simulink model "svm_dtc_winder_clean"  (R2026a)
settings: Solver=VariableStepAuto  StopTime=Tsim  MaxStep=1e-6
undefined symbols (not defined in the file): B, C_web, draw_max, draw_takeup, F0, F_ref, F_slack, ff_full, ff_on, filt_on, Fmax, h, H0, Jc, Jm, K_web, Ki_F, Ki_speed, Kp_F, Kp_speed, lambda_ref, p, r0, rc, rho, rmax, Rs, Rs_factor, T_ramp, t_rev, tau_F, Tmax, Ts_dtc, Ts_pwm, v_line_set, Vdc, w, w_max, w_min, w_ref, web_w, winder_mode_set
libraries: nesl_utility x13, fl_lib x10, ee_lib x5, slpidlib x2, eePwmGeneratorTwoLevel x1
settings Model: Creator=kunal  LastModifiedBy=kunal
settings SimscapeCC: SimscapeLogType=none

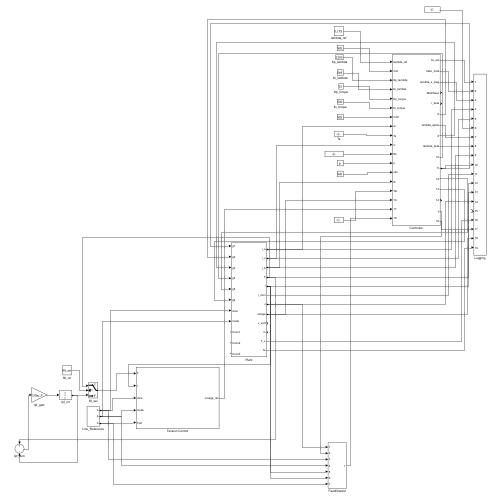
[thumbnail: Simulink's stored preview of the top-level diagram]
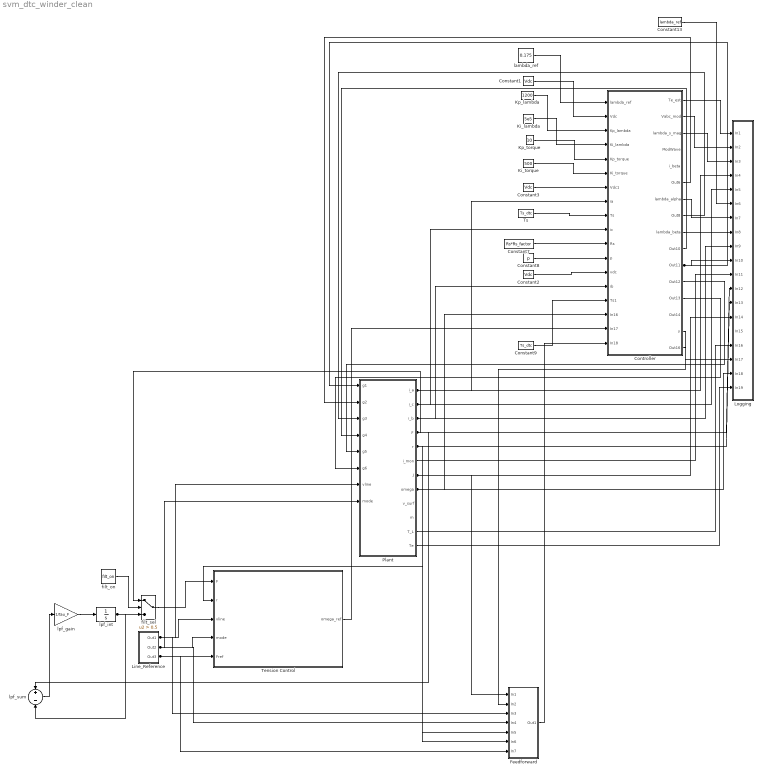
== system svm_dtc_winder_clean ==
  Constant1 : Constant  Value=Vdc
  Constant13 : Constant  Value=lambda_ref
  Constant2 : Constant  Value=Vdc
  Constant3 : Constant  Value=Vdc
  Constant7 : Constant  Value=Rs*Rs_factor
  Constant8 : Constant  Value=p
  Constant9 : Constant  Value=Ts_dtc
  Controller : Subsystem
  Feedforward : Subsystem
  Ki_lambda : Constant  Value=5e5
  Ki_torque : Constant  Value=500
  Kp_lambda : Constant  Value=1200
  Kp_torque : Constant  Value=10
  Line_Reference : Subsystem
  Logging : Subsystem
  Plant : Subsystem
  Tension Control : Subsystem
  Ts : Constant  Value=Ts_dtc
  filt_on : Constant  Value=filt_on
  filt_sel : Switch  Criteria=u2 > Threshold  Threshold=0.5  SaturateOnIntegerOverflow=off  InputSameDT=off
  lambda_ref : Constant  Value=0.175
  lpf_gain : Gain  Gain=1/tau_F
  lpf_int : Integrator  InitialCondition=F0
  lpf_sum : Sum  Inputs=+-
  wires:
  lpf_sum/1 -> lpf_gain/1
  Line_Reference/1(Out1) -> Plant/7(vline), Tension Control/3(vline), Feedforward/3(In3)
  Ki_lambda/1 -> Controller/4(Ki_lambda)
  Kp_lambda/1 -> Controller/3(Kp_lambda)
  lpf_int/1 -> lpf_sum/2, filt_sel/3
  Feedforward/1(Out1) -> Controller/18(In18)
  Constant2/1 -> Controller/13(vdc)
  Constant1/1 -> Controller/2(Vdc)
  lpf_gain/1 -> lpf_int/1
  filt_on/1 -> filt_sel/2
  lambda_ref/1 -> Controller/1(lambda_ref)
  Line_Reference/3(Out3) -> Feedforward/7(In7), Tension Control/5(Fref)
  Controller/12(Out12) -> Plant/5(g5)
  filt_sel/1 -> Tension Control/1(F)
  Line_Reference/2(Out2) -> Feedforward/4(In4), Plant/8(mode), Tension Control/4(mode)
  Tension Control/1(omega_ref) -> Controller/17(In17)
  Plant/5(r) -> Tension Control/2(r), Feedforward/5(In5), Feedforward/6(In6), Logging/13(In13)
  Plant/1(i_a) -> Controller/8(ia), Logging/4(In4)
  Plant/6(i_mon) -> Logging/11(In11)
  Plant/2(i_c) -> Logging/5(In5), Controller/10(ic)
  Plant/11(T_L) -> Logging/16(In16)
  Plant/7(J) -> Logging/14(In14), Feedforward/1(In1)
  Plant/3(i_b) -> Logging/9(In9), Controller/14(ib)
  Controller/9(lambda_beta) -> Logging/8(In8)
  Plant/12(Te) -> Logging/19(In19)
  Plant/8(omega) -> Logging/18(In18), Controller/16(In16)
  Plant/4(F) -> lpf_sum/1, filt_sel/1, Logging/12(In12)
  Ki_torque/1 -> Controller/6(Ki_torque)
  Kp_torque/1 -> Controller/5(Kp_torque)
  Controller/8(Out8) -> Plant/3(g3)
  Constant13/1 -> Logging/6(In6)
  Constant3/1 -> Controller/7(Vdc1)
  Ts/1 -> Controller/9(Ts)
  Constant9/1 -> Controller/15(Ts1)
  Constant7/1 -> Controller/11(Rs)
  Constant8/1 -> Controller/12(p)
  Controller/1(Te_est) -> Logging/1(In1)
  Controller/2(Vabc_mod) -> Logging/2(In2)
  Controller/3(lambda_s_mag) -> Logging/3(In3)
  Controller/6(Out6) -> Plant/2(g2)
  Controller/7(lambda_alpha) -> Logging/7(In7)
  Controller/10(Out10) -> Plant/4(g4)
  Controller/11(Out11) -> Plant/1(g1), Logging/10(In10)
  Controller/13(Out13) -> Plant/6(g6)
  Controller/15(y) -> Logging/17(In17)
  Controller/16(Out16) -> Feedforward/2(In2)

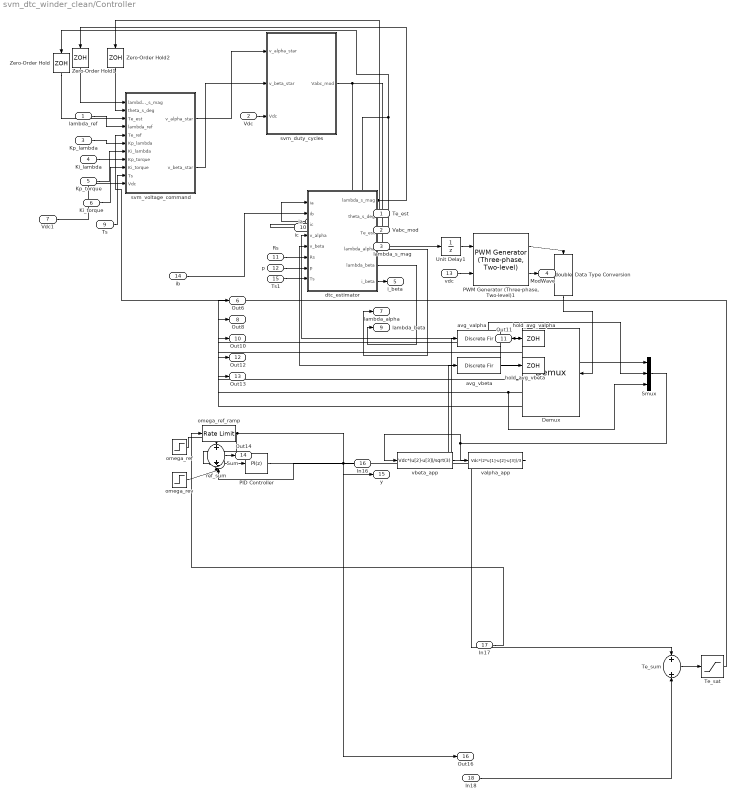
== system svm_dtc_winder_clean/Controller ==
  lambda_ref : Inport
  Vdc : Inport  Port=2
  Kp_lambda : Inport  Port=3
  Ki_lambda : Inport  Port=4
  Kp_torque : Inport  Port=5
  Ki_torque : Inport  Port=6
  Vdc1 : Inport  Port=7
  ia : Inport  Port=8
  Ts : Inport  Port=9
  ic : Inport  Port=10
  Rs : Inport  Port=11
  p : Inport  Port=12
  vdc : Inport  Port=13
  ib : Inport  Port=14
  Ts1 : Inport  Port=15
  In16 : Inport  Port=16
  In17 : Inport  Port=17
  In18 : Inport  Port=18
  Data Type Conversion : DataTypeConversion  OutDataTypeStr=double  SaturateOnIntegerOverflow=off  RndMeth=Floor
  Demux : Demux  Outputs=6
  PID Controller : slpidlib/PID Controller  Controller=PI  Form=Parallel  TimeDomain=Discrete-time  UseExternalTs=off  SampleTime=Ts_dtc  IntegratorMethod=Forward Euler  FilterMethod=Forward Euler  ControllerParametersSource=internal  P=Kp_speed  I=Ki_speed  UseKiTs=off  D=0  UseExternalDerivativeSource=off  N=100  UseFilter=on  TunerSelectOption=Transfer Function Based (PID Tuner App)  InitialConditionSource=internal  InitialConditionForIntegrator=0  InitialConditionForFilter=0  DifferentiatorICPrevScaledInput=0  ExternalReset=none  TrackingMode=off  Kt=1  LimitOutput=on  SatLimitsSource=internal  UpperSaturationLimit=5  LowerSaturationLimit=-5  LinearizeAsGain=on  AntiWindupMode=clamping  Kb=1  LimitIntegrator=off  UpperIntegratorSaturationLimit=inf  LowerIntegratorSaturationLimit=-inf  POutMin=[]  POutMax=[]  IOutMin=[]  IOutMax=[]  DOutMin=[]  DOutMax=[]  NOutMin=[]  NOutMax=[]  SumOutMin=[]  SumOutMax=[]  SaturationOutMin=[]  SaturationOutMax=[]  PParamMin=[]  PParamMax=[]  IParamMin=[]  IParamMax=[]  DParamMin=[]  DParamMax=[]  NParamMin=[]  NParamMax=[]  KbParamMin=[]  KbParamMax=[]  KtParamMin=[]  KtParamMax=[]  KbOutMin=[]  KbOutMax=[]  KtOutMin=[]  KtOutMax=[]  IntegratorOutMin=[]  IntegratorOutMax=[]  FilterOutMin=[]  FilterOutMax=[]  SumI1OutMin=[]  SumI1OutMax=[]  SumI2OutMin=[]  SumI2OutMax=[]  SumI3OutMin=[]  SumI3OutMax=[]  SumI4OutMin=[]  SumI4OutMax=[]  SumDOutMin=[]  SumDOutMax=[]  DifferentiatorOutMin=[]  DifferentiatorOutMax=[]  FilterDiffOutCoefMin=[]  FilterDiffOutCoefMax=[]  ReciprocalOutMin=[]  ReciprocalOutMax=[]  SumDenOutMin=[]  SumDenOutMax=[]  SumNumOutMin=[]  SumNumOutMax=[]  DivideOutMin=[]  DivideOutMax=[]  UdiffTsProdOutMin=[]  UdiffTsProdOutMax=[]  NTsProdOutMin=[]  NTsProdOutMax=[]  UintegralTsProdOutMin=[]  UintegralTsProdOutMax=[]  UngainTsProdOutMin=[]  UngainTsProdOutMax=[]  ClampingZeroOutDataTypeStr=Inherit: Inherit via back propagation  ClampingZeroOutMin=[]  ClampingZeroOutMax=[]  FilterDenConstantOutDataTypeStr=Inherit: Inherit via back propagation  FilterDenConstantOutMin=[]  FilterDenConstantOutMax=[]  PCopyOutDataTypeStr=Inherit: Inherit via back propagation  PCopyOutMin=[]  PCopyOutMax=[]  NCopyOutDataTypeStr=Inherit: Inherit via back propagation  NCopyOutMin=[]  NCopyOutMax=[]  IntegratorContinuousStateAttributes=''  IntegratorStateMustResolveToSignalObject=off  IntegratorRTWStateStorageClass=Auto  FilterContinuousStateAttributes=''  FilterStateMustResolveToSignalObject=off  FilterRTWStateStorageClass=Auto  ParallelPVariant=InternalParameters  IdealPVariant=Disabled  IVariant=InternalParameters  DVariant=Disabled  IntegratorVariant=Discrete  SatVariant=Enabled  AWVariant=DiscClampingParallel  PCopyVariant=Disabled  TRVariant=Disabled  FdbkBlocksVariant=Forward  IdealPFdbkVariant=Disabled  SatFdbkVariant=Disabled  DerivativeFilterVariant=Disabled  NVariant=Disabled  NCopyVariant=Disabled_SignalSpec  FilterICVariant=Disabled  IntegratorICVariant=InternalICs  ExternalResetVariant=Disabled  TRSumVariant=Passthrough  SumFdbkVariant=Disabled  SumVariant=Sum_PI  TsampFilterVariant=InternalTs  TsampNgainVariant=Passthrough  TsampIntegralVariant=Disabled_SignalSpec  ExternalSaturationOutDataTypeStr=Inherit: Same as second input  DerivativeSourceVariant=Disabled  PreIntVariant=InternalPreInt
  "PWM Generator (Three-phase, Two-level)1" : eePwmGeneratorTwoLevel/PWM Generator (Three-phase, Two-level)  PWMMode=Continuous PWM (CPWM)  CPWMMode=SPWM: sinusoidal PWM  DPWMMode=60 DPWM: 60 degree discontinuous PWM  fsw=5000  Ts=Ts_pwm
      settings: LibrarySourceBlock=|
      | ee_sl_lib/Pulse Width
      | Modulation/PWM Generator
      | (Three-phase, Two-level)
  Smux : Mux  Inputs=3
  Sum : Sum  Inputs=|+-
  Te_sat : Saturate  UpperLimit=Tmax  LowerLimit=-Tmax
  Te_sum : Sum
  Unit Delay1 : UnitDelay  SampleTime=Ts_dtc
  Zero-Order Hold : ZeroOrderHold  SampleTime=Ts_dtc
  Zero-Order Hold1 : ZeroOrderHold  SampleTime=Ts_dtc
  Zero-Order Hold2 : ZeroOrderHold  SampleTime=Ts_dtc
  avg_valpha : DiscreteFir  Coefficients=ones(1,round(Ts_dtc/Ts_pwm))/round(Ts_dtc/Ts_pwm)  SampleTime=Ts_pwm
  avg_vbeta : DiscreteFir  Coefficients=ones(1,round(Ts_dtc/Ts_pwm))/round(Ts_dtc/Ts_pwm)  SampleTime=Ts_pwm
  dtc_estimator : MATLAB Function  TreatAsAtomicUnit=on  SystemSampleTime=Ts_dtc
  hold_avg_valpha : ZeroOrderHold  SampleTime=Ts_dtc
  hold_avg_vbeta : ZeroOrderHold  SampleTime=Ts_dtc
  omega_ref : Step  Time=0.05  FinalValue=w_ref  SampleTime=Ts_dtc
  omega_ref_ramp : RateLimiter  RisingSlewLimit=700  FallingSlewLimit=-700  SampleTimeMode=inherited
  omega_rev : Step  Time=t_rev  FinalValue=-2*w_ref  SampleTime=Ts_dtc
  ref_sum : Sum
  svm_duty_cycles : MATLAB Function  TreatAsAtomicUnit=on  SystemSampleTime=Ts_dtc
  svm_voltage_command : MATLAB Function  TreatAsAtomicUnit=on  SystemSampleTime=Ts_dtc
  valpha_app : Fcn  Expr=Vdc*(2*u[1]-u[2]-u[3])/3
  vbeta_app : Fcn  Expr=Vdc*(u[2]-u[3])/sqrt(3)
  Te_est : Outport
  Vabc_mod : Outport  Port=2
  lambda_s_mag : Outport  Port=3
  ModWave : Outport  Port=4
  i_beta : Outport  Port=5
  Out6 : Outport  Port=6
  lambda_alpha : Outport  Port=7
  Out8 : Outport  Port=8
  lambda_beta : Outport  Port=9
  Out10 : Outport  Port=10
  Out11 : Outport  Port=11
  Out12 : Outport  Port=12
  Out13 : Outport  Port=13
  Out14 : Outport  Port=14
  y : Outport  Port=15
  Out16 : Outport  Port=16
  wires:
  hold_avg_valpha/1 -> dtc_estimator/4(v_alpha)
  Sum/1 -> PID Controller/1
  Demux/3 -> Out6/1, Smux/2
  In16/1 -> Sum/2
  hold_avg_vbeta/1 -> dtc_estimator/5(v_beta)
  valpha_app/1 -> avg_valpha/1
  vbeta_app/1 -> avg_vbeta/1
  ic/1 -> dtc_estimator/3(ic)
  PID Controller/1 -> y/1, Te_sum/1
  Smux/1 -> vbeta_app/1, valpha_app/1
  Zero-Order Hold/1 -> svm_voltage_command/3(Te_est)
  Data Type Conversion/1 -> Demux/1
  svm_voltage_command/2(v_beta_star) -> svm_duty_cycles/2(v_beta_star)
  dtc_estimator/1(lambda_s_mag) -> lambda_s_mag/1, Zero-Order Hold1/1
  lambda_ref/1 -> svm_voltage_command/4(lambda_ref)
  Demux/5 -> Out12/1, Smux/3
  svm_duty_cycles/1(Vabc_mod) -> Vabc_mod/1, Unit Delay1/1
  ia/1 -> dtc_estimator/1(ia)
  Te_sat/1 -> svm_voltage_command/5(Te_ref)
  dtc_estimator/2(theta_s_deg) -> Zero-Order Hold2/1
  Ki_torque/1 -> svm_voltage_command/9(Ki_torque)
  Zero-Order Hold1/1 -> svm_voltage_command/1(lambda_s_mag)
  dtc_estimator/3(Te_est) -> Te_est/1, Zero-Order Hold/1
  omega_ref_ramp/1 -> Out16/1, Sum/1
  "PWM Generator (Three-phase, Two-level)1"/1 -> Data Type Conversion/1
  avg_valpha/1 -> hold_avg_valpha/1
  p/1 -> dtc_estimator/7(p)
  svm_voltage_command/1(v_alpha_star) -> svm_duty_cycles/1(v_alpha_star)
  Zero-Order Hold2/1 -> svm_voltage_command/2(theta_s_deg)
  Ki_lambda/1 -> svm_voltage_command/7(Ki_lambda)
  In18/1 -> Te_sum/2
  dtc_estimator/6(i_beta) -> i_beta/1
  dtc_estimator/4(lambda_alpha) -> lambda_alpha/1
  omega_ref/1 -> ref_sum/1
  omega_rev/1 -> ref_sum/2
  Unit Delay1/1 -> "PWM Generator (Three-phase, Two-level)1"/1
  Te_sum/1 -> Te_sat/1
  Demux/2 -> Out8/1
  Ts1/1 -> dtc_estimator/8(Ts)
  Demux/6 -> Out13/1
  Vdc1/1 -> svm_voltage_command/11(Vdc)
  avg_vbeta/1 -> hold_avg_vbeta/1
  Demux/1 -> Smux/1, Out11/1
  In17/1 -> omega_ref_ramp/1
  Demux/4 -> Out10/1
  Rs/1 -> dtc_estimator/6(Rs)
  Kp_lambda/1 -> svm_voltage_command/6(Kp_lambda)
  ib/1 -> dtc_estimator/2(ib)
  ref_sum/1 -> Out14/1
  Kp_torque/1 -> svm_voltage_command/8(Kp_torque)
  dtc_estimator/5(lambda_beta) -> lambda_beta/1
  "PWM Generator (Three-phase, Two-level)1"/2 -> ModWave/1
  Vdc/1 -> svm_duty_cycles/3(Vdc)
  vdc/1 -> "PWM Generator (Three-phase, Two-level)1"/2
  Ts/1 -> svm_voltage_command/10(Ts)

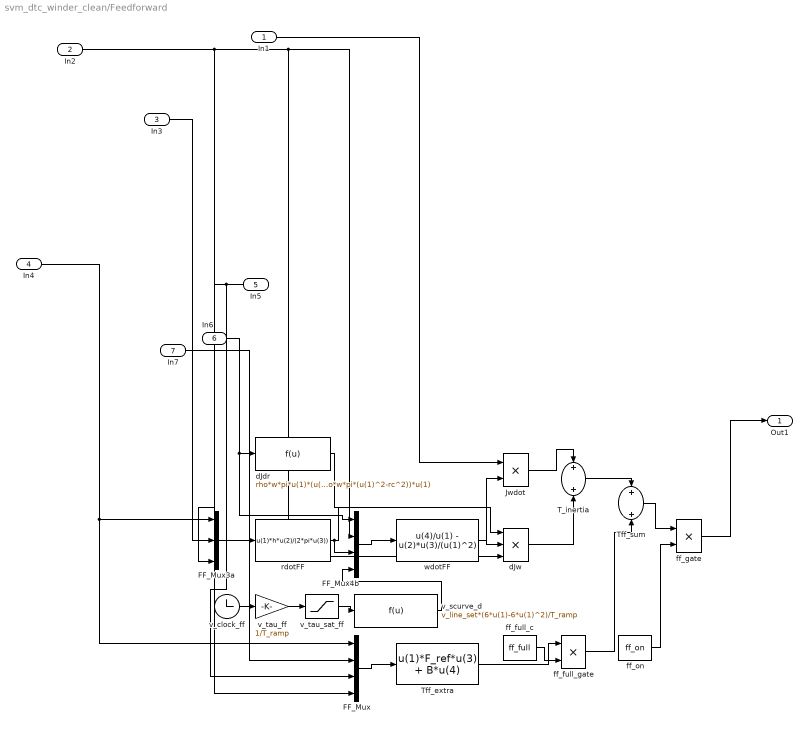
== system svm_dtc_winder_clean/Feedforward ==
  In1 : Inport
  In2 : Inport  Port=2
  In3 : Inport  Port=3
  In4 : Inport  Port=4
  In5 : Inport  Port=5
  In6 : Inport  Port=6
  In7 : Inport  Port=7
  FF_Mux : Mux
  FF_Mux3a : Mux  Inputs=3
  FF_Mux4b : Mux
  Jwdot : Product
  T_inertia : Sum
  Tff_extra : Fcn  Expr=u(1)*F_ref*u(3) + B*u(4)
  Tff_sum : Sum
  dJdr : Fcn  Expr=rho*w*pi*u(1)*(u(1)^2+rc^2) + (rho*w*pi*(u(1)^2-rc^2))*u(1)
  dJw : Product  Inputs=3
  ff_full_c : Constant  Value=ff_full
  ff_full_gate : Product
  ff_gate : Product
  ff_on : Constant  Value=ff_on
  rdotFF : Fcn  Expr=u(1)*h*u(2)/(2*pi*u(3))
  v_clock_ff : Clock
  v_scurve_d : Fcn  Expr=v_line_set*(6*u(1)-6*u(1)^2)/T_ramp
  v_tau_ff : Gain  Gain=1/T_ramp
  v_tau_sat_ff : Saturate  UpperLimit=1  LowerLimit=0
  wdotFF : Fcn  Expr=u(4)/u(1) - u(2)*u(3)/(u(1)^2)
  Out1 : Outport
  wires:
  rdotFF/1 -> FF_Mux4b/3, dJw/2
  v_tau_sat_ff/1 -> v_scurve_d/1
  In6/1 -> dJdr/1, FF_Mux4b/1
  FF_Mux4b/1 -> wdotFF/1
  FF_Mux3a/1 -> rdotFF/1
  T_inertia/1 -> Tff_sum/1
  In5/1 -> FF_Mux3a/3, FF_Mux/3
  v_scurve_d/1 -> FF_Mux4b/4
  Tff_sum/1 -> ff_gate/1
  v_clock_ff/1 -> v_tau_ff/1
  dJw/1 -> T_inertia/2
  ff_full_c/1 -> ff_full_gate/2
  v_tau_ff/1 -> v_tau_sat_ff/1
  ff_on/1 -> ff_gate/2
  In4/1 -> FF_Mux3a/1, FF_Mux/1
  Jwdot/1 -> T_inertia/1
  Tff_extra/1 -> ff_full_gate/1
  dJdr/1 -> dJw/1
  FF_Mux/1 -> Tff_extra/1
  wdotFF/1 -> Jwdot/2
  ff_full_gate/1 -> Tff_sum/2
  In3/1 -> FF_Mux3a/2
  In1/1 -> Jwdot/1
  In7/1 -> FF_Mux/2
  ff_gate/1 -> Out1/1
  In2/1 -> FF_Mux4b/2, dJw/3, FF_Mux/4

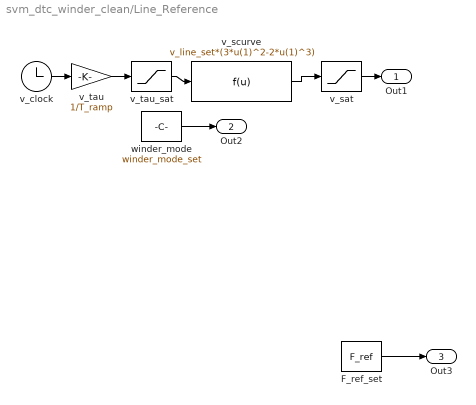
== system svm_dtc_winder_clean/Line_Reference ==
  F_ref_set : Constant  Value=F_ref
  v_clock : Clock
  v_sat : Saturate  UpperLimit=v_line_set  LowerLimit=0
  v_scurve : Fcn  Expr=v_line_set*(3*u(1)^2-2*u(1)^3)
  v_tau : Gain  Gain=1/T_ramp
  v_tau_sat : Saturate  UpperLimit=1  LowerLimit=0
  winder_mode : Constant  Value=winder_mode_set
  Out1 : Outport
  Out2 : Outport  Port=2
  Out3 : Outport  Port=3
  wires:
  v_sat/1 -> Out1/1
  v_tau_sat/1 -> v_scurve/1
  v_scurve/1 -> v_sat/1
  v_clock/1 -> v_tau/1
  v_tau/1 -> v_tau_sat/1
  winder_mode/1 -> Out2/1
  F_ref_set/1 -> Out3/1

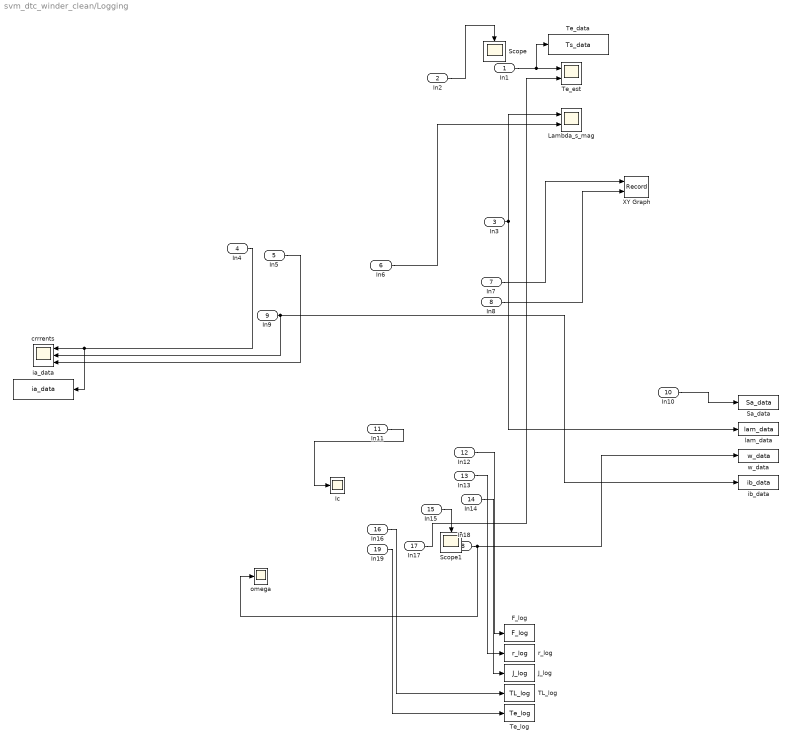
== system svm_dtc_winder_clean/Logging ==
  In1 : Inport
  In2 : Inport  Port=2
  In3 : Inport  Port=3
  In4 : Inport  Port=4
  In5 : Inport  Port=5
  In6 : Inport  Port=6
  In7 : Inport  Port=7
  In8 : Inport  Port=8
  In9 : Inport  Port=9
  In10 : Inport  Port=10
  In11 : Inport  Port=11
  In12 : Inport  Port=12
  In13 : Inport  Port=13
  In14 : Inport  Port=14
  In15 : Inport  Port=15
  In16 : Inport  Port=16
  In17 : Inport  Port=17
  In18 : Inport  Port=18
  In19 : Inport  Port=19
  F_log : ToWorkspace  VariableName=F_log  SaveFormat=Timeseries  SampleTime=-1
  Ic : Scope
      settings: ActiveDisplayYMinimum=-1.574268599657235  ActiveDisplayYMaximum=1.0954007787431075  DataLoggingVariableName=ScopeData3
  J_log : ToWorkspace  VariableName=J_log  SaveFormat=Timeseries  SampleTime=-1
  Lambda_s_mag : Scope  NumInputPorts=2
      settings: ActiveDisplayYMinimum=0.17481535622164487  ActiveDisplayYMaximum=0.1750205159753728
  Sa_data : ToWorkspace  VariableName=Sa_data  SaveFormat=Timeseries  SampleTime=-1
  Scope : Scope
      settings: ActiveDisplayYMinimum=-2.148644991246897  ActiveDisplayYMaximum=1.4968884785791123  DataLoggingVariableName=ScopeData4
  Scope1 : Scope
      settings: DataLoggingVariableName=ScopeData5
  TL_log : ToWorkspace  VariableName=TL_log  SaveFormat=Timeseries  SampleTime=-1
  Te_data : ToWorkspace  VariableName=Ts_data  SaveFormat=Timeseries  SampleTime=-1
  Te_est : Scope  NumInputPorts=2
      settings: ActiveDisplayYMinimum=-0.9384209187491952  ActiveDisplayYMaximum=5.6598245465276884
  Te_log : ToWorkspace  VariableName=Te_log  SaveFormat=Timeseries  SampleTime=-1
  XY Graph : Record  NumPorts=2.0  FileSettingsInternal="{\"entries\":[{\"content\":{\"excelSettings\":{\"content\":{},\"type\":\"Streamout.ExcelSettings\"},\"parquetSettings\":{\"content\":{},\"type\":\"Streamout.ParquetSettings\"}},\"type\":\"Streamout.FileSettingStorage\",\"uuid\":\"\"}],\"packageUris\":[\"http:\\/\\/schema.mathworks.com\\/mf0\\/streamout_blocks\\/R2020a\"],\"version\":\"1.0\"}"  FrameSettings=[0, 0]  Layout=[1 1]  SignalsInternal="{\"entries\":[{\"content\":{\"signals\":[{\"content\":{\"blockPath\":[],\"dimensions\":[1],\"domain\":\"\",\"lineColor\":\"#a2142f\",\"lineWidth\":2,\"plots\":[ 1 ],\"port\":1,\"signalID\":1,\"signalName\":\"dtc_estimator:4\"},\"type\":\"RecordBlkView.Signal\",\"uuid\":\"\"},{\"content\":{\"blockPath\":[],\"dimensions\":[1],\"domain\":\"\",\"lineColor\":\"#139fff\",\"lineWidth\":2,\"plots\":[ 1 ],\"port\":2,\"signalID\":2,\"signalName\":\"dtc_estimator:5\"},\"type\":\"RecordBlkView.Signal\",\"uuid\":\"\"}]},\"type\":\"RecordBlkView.InputSignals\",\"uuid\":\"\"}],\"packageUris\":[\"http:\\/\\/schema.mathworks.com\\/mf0\\/streamout_blocks\\/R2020a\"],\"version\":\"1.0\"}"  VisualizationBindings="{\"xyplotplugin\":{\"info\":[{\"series\":[{\"bindingParametersList\":[{\"parameter\":\"X-Axis\",\"signalID\":2,\"signalName\":\"dtc_estimator:5\"},{\"parameter\":\"Y-Axis\",\"signalID\":1,\"signalName\":\"dtc_estimator:4\"}],\"seriesID\":0}],\"subplotID\":1}]}}"  CompatibilityTag=XY
  crrrents : Scope  NumInputPorts=3
      settings: ActiveDisplayYMinimum=-0.84095457498460979  ActiveDisplayYMaximum=0.85331725762283572  DataLoggingVariableName=ScopeData13
  ia_data : ToWorkspace  VariableName=ia_data  SaveFormat=Timeseries  SampleTime=-1
  ib_data : ToWorkspace  VariableName=ib_data  SaveFormat=Timeseries  SampleTime=-1
  lam_data : ToWorkspace  VariableName=lam_data  SaveFormat=Timeseries  SampleTime=-1
  omega : Scope
      settings: ActiveDisplayYMinimum=8.40742082525544  ActiveDisplayYMaximum=24.903297754520032  DataLoggingVariableName=ScopeData2
  r_log : ToWorkspace  VariableName=r_log  SaveFormat=Timeseries  SampleTime=-1
  w_data : ToWorkspace  VariableName=w_data  SaveFormat=Timeseries  SampleTime=-1
  wires:
  In11/1 -> Ic/1
  In17/1 -> Te_est/2
  In7/1 -> XY Graph/1
  In3/1 -> Lambda_s_mag/1, lam_data/1
  In6/1 -> Lambda_s_mag/2
  In1/1 -> Te_data/1, Te_est/1
  In4/1 -> ia_data/1, crrrents/1
  In18/1 -> omega/1, w_data/1
  In16/1 -> TL_log/1
  In12/1 -> F_log/1
  In19/1 -> Te_log/1
  In10/1 -> Sa_data/1
  In9/1 -> crrrents/2, ib_data/1
  In2/1 -> Scope/1
  In5/1 -> crrrents/3
  In13/1 -> r_log/1
  In14/1 -> J_log/1
  In8/1 -> XY Graph/2
  In15/1 -> Scope1/1

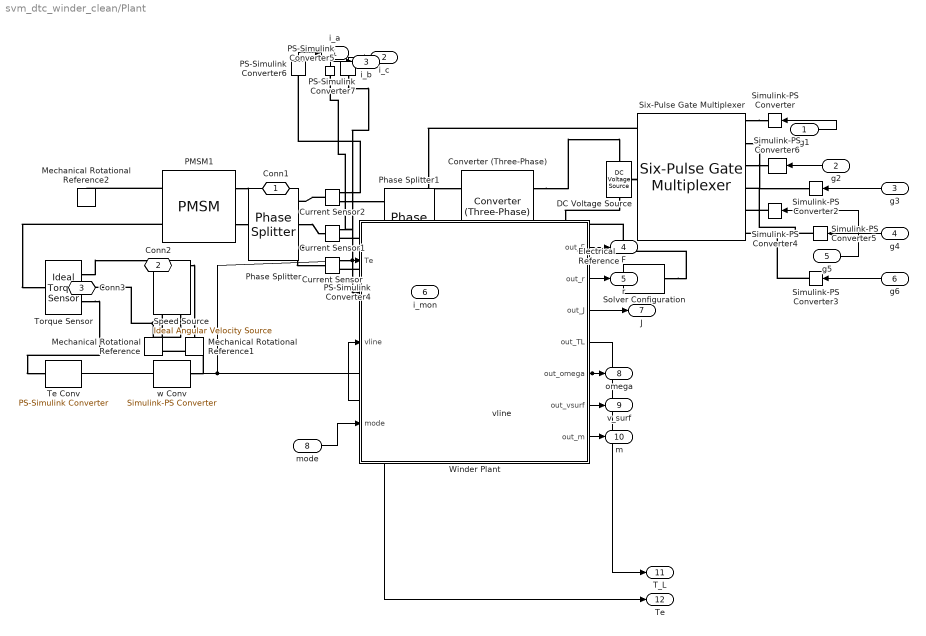
== system svm_dtc_winder_clean/Plant ==
  g1 : Inport
  g2 : Inport  Port=2
  g3 : Inport  Port=3
  g4 : Inport  Port=4
  g5 : Inport  Port=5
  g6 : Inport  Port=6
  vline : Inport  Port=7
  mode : Inport  Port=8
  Converter (Three-Phase) : ee_lib/Semiconductors & Converters/Converters/Converter (Three-Phase)  port_option=ee.enum.threePhasePort.composite  fidelity_option=ee.enum.converters.fidelity.detailed  device_type=ee.enum.converters.switchingdevice.ideal  showThermalPort=false  K=0  Vth=0.5 V  Vgt=1 V  Vgt_off=-1 V  Ih=1 A  Vf=0.8 V  Ron=0.001 Ohm  Rds=0.001 Ohm  Goff=1e-6 1/Ohm  Eon_scalar=22.86e-3 J  Eoff_scalar=17.14e-3 J  Eoff_natural_commutation=10e-3 J  Voff=300 V  Iout_scalar=600 A  onCurrentMeasDelay=0 s  useCurrentFromPreviousCycle=false  useVoltageFromPreviousCycle=false  diode_param=ee.enum.converters.protectiondiode.nodynamics  diode_Vf=0.8 V  diode_Ron=0.001 Ohm  diode_Goff=1e-5 1/Ohm  diode_C=50 nF  diode_iRM=-235 A  diode_iF=300 A  diode_idot=-50 A/us  diode_trr_param=ee.enum.converters.diodetrr.trr_factor  diode_trr_factor=3  diode_trr=15 us  diode_Qrr=1500 s*uA  diode_rec_loss_model=ee.enum.diode.reverseRecoveryModel.fixed  diode_ErecVal=0 J  diode_scaleWithIandV=false  diode_ErecMat=zeros(2, 3) J  diode_TjrecVec=[298.15, 398.15] K  diode_IfrecVec=[.1, 1, 10] A  diode_IrecVal=10 A  diode_VrecVal=10 V  diode_tFilter=1 / 1000 / 100 s  thermal_network_parameterization=ee.enum.thermalNetworkTopology.external  Rth=[.08, .5] K/W  Rth_Cauer=[.08, .1, .5] K/W  Rth_Foster=[.08, .14, .22, .16] K/W  thermal_mass_parameterization=ee.enum.thermalNetwork.timeconstant  thermal_mass=[.01, .5] J/K  thermal_mass_Cauer=[.01, .1, .5] J/K  thermal_mass_Foster=[.001, .005, .05, .5] J/K  thermal_time_constant=[.001, .2] s  thermal_time_constant_Cauer=[.001, .1, .2] s  thermal_time_constant_Foster=[7e-05, .0007, .01, .08] s  thermal_mass_initial_temperatures=[25, 25] degC  thermal_mass_initial_temperatures_Cauer=[25, 25, 25] degC  junction_thermal_mass=0.01 J/K  Tvec_initial_Foster=[25, 25, 25, 25] degC  snubber_type=ee.enum.converters.snubber.exclude  Cs=1e-7 F  Rs=0.1 Ohm  Vce_loss=[0, 150, 300] V
  Current Sensor : fl_lib/Electrical/Electrical Sensors/Current Sensor
  Current Sensor1 : fl_lib/Electrical/Electrical Sensors/Current Sensor
  Current Sensor2 : fl_lib/Electrical/Electrical Sensors/Current Sensor
  DC Voltage Source : fl_lib/Electrical/Electrical Sources/DC Voltage Source  v0=Vdc V
  Electrical Reference : fl_lib/Electrical/Electrical Elements/Electrical Reference
  Mechanical Rotational Reference : fl_lib/Mechanical/Rotational Elements/Mechanical Rotational Reference
  Mechanical Rotational Reference1 : fl_lib/Mechanical/Rotational Elements/Mechanical Rotational Reference
  Mechanical Rotational Reference2 : fl_lib/Mechanical/Rotational Elements/Mechanical Rotational Reference
  PMSM1 : ee_lib/Electromechanical/Permanent Magnet/PMSM  port_option=ee.enum.threePhasePort.composite  winding_type=ee.enum.electromech.statorconfiguration.wye  machine_param=ee.enum.pmsm.parameterization.constant  nPolePairs=p  pmflux_param=ee.enum.pmflux.fluxlinkage  pm_flux_linkage=lambda_f Wb  torque_constant=0.18 N*m/A  back_emf_constant=0.18 V*s/rad  stator_param=ee.enum.statorparam.LdLqL0  Ld=Ld H  Lq=Lq H  idVec=[-200, 0, 200] A  iqVec=[-200, 0, 200] A  LdMatrix=0.0002 * ones(3, 3) H  LqMatrix=0.0002 * ones(3, 3) H  PmMatrix=0.1 * ones(3, 3) Wb  ktMatrix=0.18 * ones(3, 3) N*m/A  keMatrix=0.18 * ones(3, 3) V*s/rad  L0=0.00016 H  Ls=0.0002 H  Lm=-0.00002 H  Ms=0.00002 H  Rs=Rs Ohm  zero_sequence=ee.enum.park.zerosequence.include  axes_param=ee.enum.rotorangle.daxis  loss_param=ee.enum.ironloss.none  losses_oc=[0, 0, 0] W  losses_sc=[0, 0, 0] W  f_losses=60 Hz  Isc_losses=95 A  J=0 kg*m^2  lam=0 N*m*s/rad  i_d_specify=off  i_d_priority=None  i_d=0 A  i_d_nominal_specify=off  i_d_nominal_value=1  i_d_nominal_unit=A  i_q_specify=off  i_q_priority=None  i_q=0 A  i_q_nominal_specify=off  i_q_nominal_value=1  i_q_nominal_unit=A  torque_specify=off  torque_priority=None  torque=0 N*m  torque_nominal_specify=off  torque_nominal_value=1  torque_nominal_unit=N*m  angular_velocity_specify=off  angular_velocity_priority=High  angular_velocity=0 rpm  angular_velocity_nominal_specify=off  angular_velocity_nominal_value=1  angular_velocity_nominal_unit=rpm  angular_position_specify=off  angular_position_priority=High  angular_position=0 deg  angular_position_nominal_specify=off  angular_position_nominal_value=1  angular_position_nominal_unit=deg  alpha=3.93e-3 1/K  alpha_flux=-0.001 1/K  Tmeas=298.15 K  stator_thermal_mass=100 J/K  rotor_thermal_mass=200 J/K  Rm_percent_rotor=90  Rd_percent_rotor=30  temperatureA_specify=off  temperatureA_priority=High  temperatureA=25 degC  temperatureA_nominal_specify=off  temperatureA_nominal_value=1  temperatureA_nominal_unit=degC  temperatureB_specify=off  temperatureB_priority=High  temperatureB=25 degC  temperatureB_nominal_specify=off  temperatureB_nominal_value=1  temperatureB_nominal_unit=degC  temperatureC_specify=off  temperatureC_priority=High  temperatureC=25 degC  temperatureC_nominal_specify=off  temperatureC_nominal_value=1  temperatureC_nominal_unit=degC  temperatureR_specify=off  temperatureR_priority=High  temperatureR=25 degC  temperatureR_nominal_specify=off  temperatureR_nominal_value=1  temperatureR_nominal_unit=degC
  PS-Simulink Converter{4..7} (4 alike) : nesl_utility/PS-Simulink Converter  PhysicalDomain=network_engine_domain  SubClassName=ps_output  LeftPortType=input  RightPortType=output  PseudoPeriodic=off  Frequencies=[]  VectorFormat=inherit  Unit=inherit  AffineConversion=off
  Phase Splitter : ee_lib/Connectors & References/Phase Splitter
  Phase Splitter1 : ee_lib/Connectors & References/Phase Splitter
  Simulink-PS Converter{,2..6} (6 alike) : nesl_utility/Simulink-PS Converter  PhysicalDomain=network_engine_domain  SubClassName=ps_input  LeftPortType=input  RightPortType=output  PseudoPeriodic=off  Frequencies=[]  NoiseDistribution=none  NoiseParameters=[]  Unit=1  AffineConversion=off  FilteringAndDerivatives=provide  SimscapeFilterOrder=1  InputFilterTimeConstant=0.001  UdotUserProvided=0
  Six-Pulse Gate Multiplexer : ee_lib/Semiconductors & Converters/Converters/Six-Pulse Gate Multiplexer  port_option=ee.enum.controlport.ps
  Solver Configuration : nesl_utility/Solver Configuration  PhysicalDomain=network_engine_domain  SubClassName=solver  LeftPortType=input  RightPortType=generic  Tones=[]  Harmonics=[]  SimulateNoise=off  Profile=off  UseLocalSampling=off  EnableSwitchedLinearOptims=on  FrequencyDomain=off  UseCCode=off  RelTol=0.001  AbsTol=0.001  MinStep=1e-09  ToWorkspace=off  RevertToSquareIcSolve=off  NumHomotopyIterations=100  PhasorMode=off  PhasorModeNumHarmonics=1  ConsistencySolver=NEWTON_XTOL_AFTER_FTOL  CanonicalOrdering=CANONICAL  OptimizeIntermediates=OPTIMIZED  IndexReductionMethod=DerivativeReplacement  DoDC=off  ResidualTolerance=1e-09  ConsistencyTolSource=GLOBAL  ConsistencyAbsTol=0.001  ConsistencyRelTol=0.001  ConsistencyTolFactor=0.001  UseLocalSolver=off  LocalSolverChoice=NE_BACKWARD_EULER_ADVANCER  ResolveIndetEquations=on  FunctionEvalNumThread=1  LocalSolverSampleTime=0.001  DoFixedCost=off  MaxNonlinIter=3  MaxModeIter=2  ComputeImpulses=off  ImpulseIterations=2  LinearAlgebra=auto  LinearAlgebraNumThread=0  EquationFormulation=NE_TIME_EF  DelaysMemoryBudget=1024  AutomaticFiltering=on  FilteringTimeConstant=0.001  PartitionStorageMethod=AS_NEEDED  PartitionMemoryBudget=1024  PartitionMethod=ROBUST  MultibodyUseLocalSolver=off  MultibodyLocalSolverChoice=ODE1  MultibodyLocalSolverSampleTime=0.001
  Speed Source : fl_lib/Mechanical/Mechanical Sources/Ideal Angular Velocity Source
  Te Conv : nesl_utility/PS-Simulink Converter  PhysicalDomain=network_engine_domain  SubClassName=ps_output  LeftPortType=input  RightPortType=output  PseudoPeriodic=off  Frequencies=[]  VectorFormat=inherit  Unit=inherit  AffineConversion=off
  Torque Sensor : fl_lib/Mechanical/Mechanical Sensors/Ideal Torque Sensor
  Winder Plant : Subsystem
  w Conv : nesl_utility/Simulink-PS Converter  PhysicalDomain=network_engine_domain  SubClassName=ps_input  LeftPortType=input  RightPortType=output  PseudoPeriodic=off  Frequencies=[]  NoiseDistribution=none  NoiseParameters=[]  Unit=1  AffineConversion=off  FilteringAndDerivatives=provide  SimscapeFilterOrder=1  InputFilterTimeConstant=0.001  UdotUserProvided=0
  Conn1 : PMIOPort  Side=Left
  Conn2 : PMIOPort  Port=2  Side=Left
  Conn3 : PMIOPort  Port=3  Side=Left
  i_a : Outport
  i_c : Outport  Port=2
  i_b : Outport  Port=3
  F : Outport  Port=4
  r : Outport  Port=5
  i_mon : Outport  Port=6
  J : Outport  Port=7
  omega : Outport  Port=8
  v_surf : Outport  Port=9
  m : Outport  Port=10
  T_L : Outport  Port=11
  Te : Outport  Port=12
  wires:
  Winder Plant/7(out_m) -> m/1
  Winder Plant/2(out_r) -> r/1
  Te Conv/1 -> Te/1, Winder Plant/1(Te)
  PS-Simulink Converter7/1 -> i_c/1
  mode/1 -> Winder Plant/3(mode)
  Winder Plant/3(out_J) -> J/1
  g6/1 -> Simulink-PS Converter3/1
  Winder Plant/4(out_TL) -> T_L/1
  g3/1 -> Simulink-PS Converter2/1
  Winder Plant/1(out_F) -> F/1
  PS-Simulink Converter6/1 -> i_a/1
  g4/1 -> Simulink-PS Converter5/1
  g5/1 -> Simulink-PS Converter4/1
  Winder Plant/5(out_omega) -> w Conv/1, omega/1
  g1/1 -> Simulink-PS Converter/1
  Winder Plant/6(out_vsurf) -> v_surf/1
  PS-Simulink Converter5/1 -> i_b/1
  PS-Simulink Converter4/1 -> i_mon/1
  g2/1 -> Simulink-PS Converter6/1
  vline/1 -> Winder Plant/2(vline)
  connections:
  Simulink-PS Converter5/RConn1 -- Six-Pulse Gate Multiplexer/LConn4
  Converter (Three-Phase)/RConn1 -- DC Voltage Source/LConn1
  Simulink-PS Converter3/RConn1 -- Six-Pulse Gate Multiplexer/LConn6
  Phase Splitter1/RConn2 -- Current Sensor1/RConn2
  Current Sensor/RConn1 -- PS-Simulink Converter7/LConn1 -- PS-Simulink Converter4/LConn1
  w Conv/RConn1 -- Speed Source/RConn1
  Converter (Three-Phase)/LConn2 -- Phase Splitter1/LConn1
  Current Sensor2/RConn2 -- Phase Splitter1/RConn1
  Electrical Reference/LConn1 -- Solver Configuration/RConn1 -- Converter (Three-Phase)/RConn2 -- DC Voltage Source/RConn1
  PMSM1/RConn2 -- Mechanical Rotational Reference2/LConn1
  Six-Pulse Gate Multiplexer/RConn1 -- Converter (Three-Phase)/LConn1
  Torque Sensor/RConn2 -- Te Conv/LConn1
  Mechanical Rotational Reference/LConn1 -- Conn3/RConn1 -- Speed Source/RConn2
  Simulink-PS Converter4/RConn1 -- Six-Pulse Gate Multiplexer/LConn5
  Current Sensor2/RConn1 -- PS-Simulink Converter6/LConn1
  Current Sensor1/RConn1 -- PS-Simulink Converter5/LConn1
  PMSM1/RConn1 -- Torque Sensor/LConn1
  Six-Pulse Gate Multiplexer/LConn2 -- Simulink-PS Converter2/RConn1
  PMSM1/LConn1 -- Phase Splitter/LConn1
  Torque Sensor/RConn1 -- Speed Source/LConn1
  Phase Splitter1/RConn3 -- Current Sensor/RConn2
  Six-Pulse Gate Multiplexer/LConn3 -- Simulink-PS Converter6/RConn1
  Six-Pulse Gate Multiplexer/LConn1 -- Simulink-PS Converter/RConn1
  Phase Splitter/RConn2 -- Current Sensor1/LConn1
  Phase Splitter/RConn3 -- Current Sensor/LConn1
  Current Sensor2/LConn1 -- Phase Splitter/RConn1
  Conn2/RConn1 -- Mechanical Rotational Reference1/LConn1
  PMSM1/LConn2 -- Conn1/RConn1

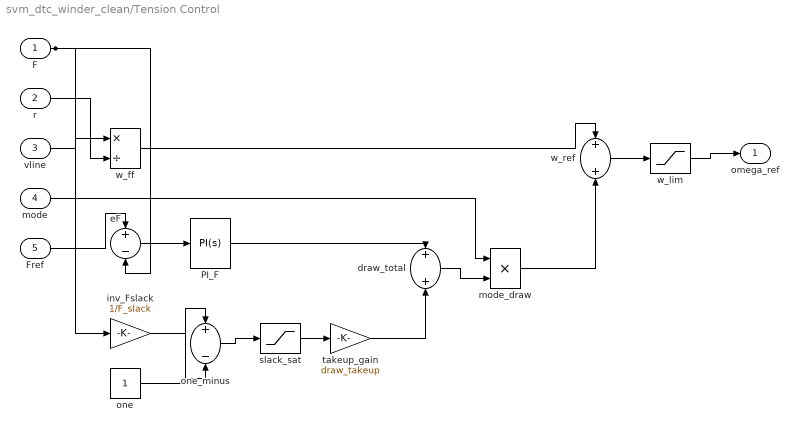
== system svm_dtc_winder_clean/Tension Control ==
  F : Inport
  r : Inport  Port=2
  vline : Inport  Port=3
  mode : Inport  Port=4
  Fref : Inport  Port=5
  PI_F : slpidlib/PID Controller  Controller=PI  Form=Parallel  TimeDomain=Continuous-time  UseExternalTs=off  SampleTime=-1  IntegratorMethod=Forward Euler  FilterMethod=Forward Euler  ControllerParametersSource=internal  P=Kp_F  I=Ki_F  UseKiTs=off  D=0  UseExternalDerivativeSource=off  N=100  UseFilter=on  TunerSelectOption=Transfer Function Based (PID Tuner App)  InitialConditionSource=internal  InitialConditionForIntegrator=0  InitialConditionForFilter=0  DifferentiatorICPrevScaledInput=0  ExternalReset=none  TrackingMode=off  Kt=1  LimitOutput=on  SatLimitsSource=internal  UpperSaturationLimit=draw_max  LowerSaturationLimit=-draw_max  LinearizeAsGain=on  AntiWindupMode=clamping  Kb=1  LimitIntegrator=off  UpperIntegratorSaturationLimit=inf  LowerIntegratorSaturationLimit=-inf  POutMin=[]  POutMax=[]  IOutMin=[]  IOutMax=[]  DOutMin=[]  DOutMax=[]  NOutMin=[]  NOutMax=[]  SumOutMin=[]  SumOutMax=[]  SaturationOutMin=[]  SaturationOutMax=[]  PParamMin=[]  PParamMax=[]  IParamMin=[]  IParamMax=[]  DParamMin=[]  DParamMax=[]  NParamMin=[]  NParamMax=[]  KbParamMin=[]  KbParamMax=[]  KtParamMin=[]  KtParamMax=[]  KbOutMin=[]  KbOutMax=[]  KtOutMin=[]  KtOutMax=[]  IntegratorOutMin=[]  IntegratorOutMax=[]  FilterOutMin=[]  FilterOutMax=[]  SumI1OutMin=[]  SumI1OutMax=[]  SumI2OutMin=[]  SumI2OutMax=[]  SumI3OutMin=[]  SumI3OutMax=[]  SumI4OutMin=[]  SumI4OutMax=[]  SumDOutMin=[]  SumDOutMax=[]  DifferentiatorOutMin=[]  DifferentiatorOutMax=[]  FilterDiffOutCoefMin=[]  FilterDiffOutCoefMax=[]  ReciprocalOutMin=[]  ReciprocalOutMax=[]  SumDenOutMin=[]  SumDenOutMax=[]  SumNumOutMin=[]  SumNumOutMax=[]  DivideOutMin=[]  DivideOutMax=[]  UdiffTsProdOutMin=[]  UdiffTsProdOutMax=[]  NTsProdOutMin=[]  NTsProdOutMax=[]  UintegralTsProdOutMin=[]  UintegralTsProdOutMax=[]  UngainTsProdOutMin=[]  UngainTsProdOutMax=[]  ClampingZeroOutDataTypeStr=Inherit: Inherit via back propagation  ClampingZeroOutMin=[]  ClampingZeroOutMax=[]  FilterDenConstantOutDataTypeStr=Inherit: Inherit via back propagation  FilterDenConstantOutMin=[]  FilterDenConstantOutMax=[]  PCopyOutDataTypeStr=Inherit: Inherit via back propagation  PCopyOutMin=[]  PCopyOutMax=[]  NCopyOutDataTypeStr=Inherit: Inherit via back propagation  NCopyOutMin=[]  NCopyOutMax=[]  IntegratorContinuousStateAttributes=''  IntegratorStateMustResolveToSignalObject=off  IntegratorRTWStateStorageClass=Auto  FilterContinuousStateAttributes=''  FilterStateMustResolveToSignalObject=off  FilterRTWStateStorageClass=Auto  ParallelPVariant=InternalParameters  IdealPVariant=Disabled  IVariant=InternalParameters  DVariant=Disabled  IntegratorVariant=Continuous  SatVariant=Enabled  AWVariant=ContClampingParallel  PCopyVariant=Disabled  TRVariant=Disabled  FdbkBlocksVariant=Forward  IdealPFdbkVariant=Disabled  SatFdbkVariant=Disabled  DerivativeFilterVariant=Disabled  NVariant=Disabled  NCopyVariant=Disabled_SignalSpec  FilterICVariant=Disabled  IntegratorICVariant=InternalICs  ExternalResetVariant=Disabled  TRSumVariant=Passthrough  SumFdbkVariant=Disabled  SumVariant=Sum_PI  TsampFilterVariant=InternalTs  TsampNgainVariant=Passthrough  TsampIntegralVariant=Disabled_SignalSpec  ExternalSaturationOutDataTypeStr=Inherit: Same as second input  DerivativeSourceVariant=Disabled  PreIntVariant=InternalPreInt
  draw_total : Sum
  eF : Sum  Inputs=+-
  inv_Fslack : Gain  Gain=1/F_slack
  mode_draw : Product
  one : Constant
  one_minus : Sum  Inputs=+-
  slack_sat : Saturate  UpperLimit=1  LowerLimit=0
  takeup_gain : Gain  Gain=draw_takeup
  w_ff : Product  Inputs=*/
  w_lim : Saturate  UpperLimit=w_max  LowerLimit=w_min
  w_ref : Sum
  omega_ref : Outport
  wires:
  vline/1 -> w_ff/1
  r/1 -> w_ff/2
  Fref/1 -> eF/1
  F/1 -> eF/2, inv_Fslack/1
  eF/1 -> PI_F/1
  inv_Fslack/1 -> one_minus/2
  one/1 -> one_minus/1
  one_minus/1 -> slack_sat/1
  slack_sat/1 -> takeup_gain/1
  PI_F/1 -> draw_total/1
  takeup_gain/1 -> draw_total/2
  mode/1 -> mode_draw/1
  draw_total/1 -> mode_draw/2
  w_ff/1 -> w_ref/1
  mode_draw/1 -> w_ref/2
  w_ref/1 -> w_lim/1
  w_lim/1 -> omega_ref/1

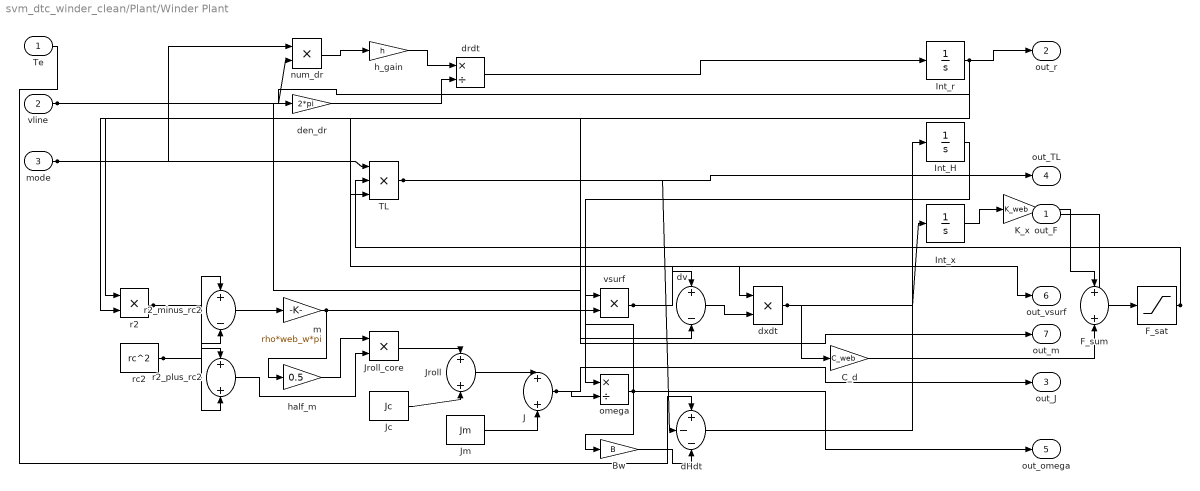
== system svm_dtc_winder_clean/Plant/Winder Plant ==
  Te : Inport
  vline : Inport  Port=2
  mode : Inport  Port=3
  Bw : Gain  Gain=B
  C_d : Gain  Gain=C_web
  F_sat : Saturate  UpperLimit=Fmax  LowerLimit=0
  F_sum : Sum
  Int_H : Integrator  InitialCondition=H0
  Int_r : Integrator  InitialCondition=r0  LimitOutput=on  UpperSaturationLimit=rmax  LowerSaturationLimit=rc
  Int_x : Integrator  InitialCondition=F0/K_web  LimitOutput=on  UpperSaturationLimit=Fmax/K_web  LowerSaturationLimit=0
  J : Sum
  Jc : Constant  Value=Jc
  Jm : Constant  Value=Jm
  Jroll : Sum
  Jroll_core : Product
  K_x : Gain  Gain=K_web
  TL : Product  Inputs=3
  dHdt : Sum  Inputs=+--
  den_dr : Gain  Gain=2*pi
  drdt : Product  Inputs=*/
  dv : Sum  Inputs=+-
  dxdt : Product
  h_gain : Gain  Gain=h
  half_m : Gain  Gain=0.5
  m : Gain  Gain=rho*web_w*pi
  num_dr : Product
  omega : Product  Inputs=*/
  r2 : Product
  r2_minus_rc2 : Sum  Inputs=+-
  r2_plus_rc2 : Sum
  rc2 : Constant  Value=rc^2
  vsurf : Product
  out_F : Outport
  out_r : Outport  Port=2
  out_J : Outport  Port=3
  out_TL : Outport  Port=4
  out_omega : Outport  Port=5
  out_vsurf : Outport  Port=6
  out_m : Outport  Port=7
  wires:
  Int_r/1 -> r2/1, r2/2, TL/3, vsurf/2, den_dr/1, out_r/1
  r2/1 -> r2_minus_rc2/1, r2_plus_rc2/1
  rc2/1 -> r2_minus_rc2/2, r2_plus_rc2/2
  r2_minus_rc2/1 -> m/1
  m/1 -> half_m/1, out_m/1
  half_m/1 -> Jroll_core/1
  r2_plus_rc2/1 -> Jroll_core/2
  Jroll_core/1 -> Jroll/1
  Jc/1 -> Jroll/2
  Jroll/1 -> J/1
  Jm/1 -> J/2
  Int_H/1 -> omega/1
  J/1 -> omega/2, out_J/1
  mode/1 -> TL/1, num_dr/1, dxdt/1
  F_sat/1 -> TL/2, out_F/1
  omega/1 -> vsurf/1, Bw/1, out_omega/1
  vline/1 -> num_dr/2, dv/2
  num_dr/1 -> h_gain/1
  h_gain/1 -> drdt/1
  den_dr/1 -> drdt/2
  Te/1 -> dHdt/1
  TL/1 -> dHdt/2, out_TL/1
  Bw/1 -> dHdt/3
  vsurf/1 -> dv/1, out_vsurf/1
  dv/1 -> dxdt/2
  drdt/1 -> Int_r/1
  dHdt/1 -> Int_H/1
  dxdt/1 -> Int_x/1, C_d/1
  Int_x/1 -> K_x/1
  K_x/1 -> F_sum/1
  C_d/1 -> F_sum/2
  F_sum/1 -> F_sat/1

== matlab function svm_dtc_winder_clean/Controller/svm_voltage_command ==
  settings: updateMethod=DISCRETE
  data: lambda_s_mag input; v_alpha_star output; theta_s_deg input; Te_est input; lambda_ref input; Te_ref input; Kp_lambda input; Ki_lambda input; Kp_torque input; Ki_torque input; Ts input; v_beta_star output; Vdc input
function [v_alpha_star, v_beta_star] = svm_voltage_command(lambda_s_mag, theta_s_deg, Te_est, ...
    lambda_ref, Te_ref, Kp_lambda, Ki_lambda, Kp_torque, Ki_torque, Ts, Vdc)
%#codegen
% SVM-DTC voltage command generator (Part 5.2), WITH ANTI-WINDUP.
%
% Two PI controllers act in a frame aligned with the stator flux vector
% (the "M-T frame": M = along flux, T = 90 deg ahead of flux). Each PI's
% unsaturated output is clamped to the max voltage the inverter can
% actually deliver (Vdc/sqrt(3), linear modulation region), and the
% integrator only accumulates when doing so would NOT push the output
% further past that limit (clamping/conditional anti-windup). Without
% this, once svm_duty_cycles saturates Vabc_mod to +/-1, the real
% applied voltage stops tracking the command, the flux/torque error
% stops shrinking, and the integrators wind up without bound -- which
% is exactly the growing-oscillation-then-permanent-saturation behavior
% seen without this fix.
%
% Inputs:
%   lambda_s_mag, theta_s_deg, Te_est - from dtc_estimator, unchanged
%   lambda_ref, Te_ref                - references, unchanged
%   Kp_lambda, Ki_lambda              - flux PI gains
%   Kp_torque, Ki_torque              - torque PI gains
%   Ts                                 - sample time [s]
%   Vdc                                - DC bus voltage [V] (new input --
%                                        wire your existing Vdc constant
%                                        into a new 11th input port here)
%
% Outputs:
%   v_alpha_star, v_beta_star - desired stator voltage vector in the
%                               stationary alpha-beta frame [V]

persistent int_lambda int_torque
if isempty(int_lambda)
    int_lambda = 0;
    int_torque = 0;
end

Vmax = Vdc / sqrt(3);   % max achievable voltage magnitude per M/T axis,
                        % linear (non-overmodulated) region

%% --- Flux PI (M-axis voltage command), with anti-windup ---
err_lambda   = lambda_ref - lambda_s_mag;
v_M_unsat    = Kp_lambda * err_lambda + Ki_lambda * int_lambda;
v_M_star     = min(max(v_M_unsat, -Vmax), Vmax);
% Conditional integration: only accumulate if not saturated, or if
% accumulating would pull the output back toward the unsaturated range.
if (v_M_star == v_M_unsat) || (err_lambda * (v_M_unsat - v_M_star) < 0)
    int_lambda = int_lambda + Ts * err_lambda;
end

%% --- Torque PI (T-axis voltage command), with anti-windup ---
err_torque   = Te_ref - Te_est;
v_T_unsat    = Kp_torque * err_torque + Ki_torque * int_torque;
v_T_star     = min(max(v_T_unsat, -Vmax), Vmax);
if (v_T_star == v_T_unsat) || (err_torque * (v_T_unsat - v_T_star) < 0)
    int_torque = int_torque + Ts * err_torque;
end

%% --- Rotate M-T command back into stationary alpha-beta frame ---
% (inverse rotation by the stator flux angle theta_s, Part 5.2)
theta_s_rad  = theta_s_deg * pi/180;
v_alpha_star = v_M_star*cos(theta_s_rad) - v_T_star*sin(theta_s_rad);
v_beta_star  = v_M_star*sin(theta_s_rad) + v_T_star*cos(theta_s_rad);

end

== matlab function svm_dtc_winder_clean/Controller/dtc_estimator ==
  settings: updateMethod=DISCRETE
  data: ia input; lambda_s_mag output; ib input; ic input; v_alpha input; v_beta input; Rs input; p input; Ts input; theta_s_deg output; Te_est output; lambda_alpha output; lambda_beta output; i_beta output
function [lambda_s_mag, theta_s_deg, Te_est, lambda_alpha, lambda_beta, i_beta] = dtc_estimator(ia, ib, ic, v_alpha, v_beta, Rs, p, Ts)
%#codegen
% DTC flux and torque estimator (voltage model, Part 4.3)
% Implements this as a MATLAB Function block with two persistent
% integrator states (lambda_alpha, lambda_beta).
%
% Inputs:
%   ia, ib, ic      - measured phase currents [A]
%   v_alpha, v_beta - inverter output voltage in alpha-beta frame [V]
%                     (computed upstream from the switching state, Part 3.2)
%   Rs              - stator resistance [ohm]
%   p               - pole pairs
%   Ts              - sample time [s]
%
% Outputs:
%   lambda_s_mag - stator flux magnitude [Wb]
%   theta_s_deg  - stator flux angle [deg], wrapped to [0,360)
%   Te_est       - estimated electromagnetic torque [N*m]
%   lambda_alpha, lambda_beta - flux components, useful for scope/debug

%{
This is the block that answers the two questions torque control actually depends on: how big is my stator flux, and what angle is it 
at relative to where it started — recall from Part 4.2, torque depends on the angle between stator flux and rotor flux, 
and this angle is embedded in how theta_s_deg evolves over time.
%}


persistent lam_a lam_b
if isempty(lam_a)
    lam_a = 0.175;
    lam_b = 0;
end
%% Correct physical current inversion from the sensors
ia_true = -ia;
ib_true = -ib;

%% Clarke transform of true currents
i_alpha = ia_true;
i_beta  = (1/sqrt(3))*ia_true + (2/sqrt(3))*ib_true;

%% Flux integration (Part 4.3) — forward Euler, simplest form
% NOTE: pure integration drifts at low speed (Problem 3, Part 5.1).
% Once this base version works, replace with a low-pass-filter-based
% or closed-loop observer estimator and compare.
lam_a = lam_a + Ts * (v_alpha - Rs*i_alpha);
lam_b = lam_b + Ts * (v_beta  - Rs*i_beta);


lambda_alpha = lam_a;
lambda_beta  = lam_b;

%% Magnitude and angle
lambda_s_mag = sqrt(lam_a^2 + lam_b^2);
theta_s_rad  = atan2(lam_b, lam_a);
theta_s_deg  = mod(theta_s_rad * 180/pi, 360);

%% Torque estimate (Part 4.3)
Te_est = 1.5 * p * (lam_a*i_beta - lam_b*i_alpha);

end

== matlab function svm_dtc_winder_clean/Controller/svm_duty_cycles ==
  settings: updateMethod=DISCRETE
  data: v_alpha_star input; Vabc_mod output; v_beta_star input; Vdc input
function Vabc_mod = svm_duty_cycles(v_alpha_star, v_beta_star, Vdc)
%#codegen
% Converts desired alpha-beta voltages into a 3-phase normalized 
% modulating vector for the Simulink PWM Generator block.

%% Inverse Clarke: alpha-beta -> three-phase reference voltages
v_a = v_alpha_star;
v_b = -0.5*v_alpha_star + (sqrt(3)/2)*v_beta_star;
v_c = -0.5*v_alpha_star - (sqrt(3)/2)*v_beta_star;

%% Min-max common-mode injection (SVPWM equivalent)
v_max = max([v_a, v_b, v_c]);
v_min = min([v_a, v_b, v_c]);
v_offset = 0.5*(v_max + v_min);

v_a_mod = v_a - v_offset;
v_b_mod = v_b - v_offset;
v_c_mod = v_c - v_offset;

%% Output in VOLTS (PWM Generator normalises by Vdc/2 itself)
Vabc_mod = [v_a_mod; v_b_mod; v_c_mod];

%% Saturate to the inverter limit
Vabc_mod = min(max(Vabc_mod, -Vdc/2), Vdc/2);
